simulink model "SIL_PID_vs_LeadLag"  (R2026a)
settings: Solver=VariableStepAuto
libraries: simulink_extras x14, simulink x4, slpidlib x2
settings Model: Creator=jamie  LastModifiedBy=root

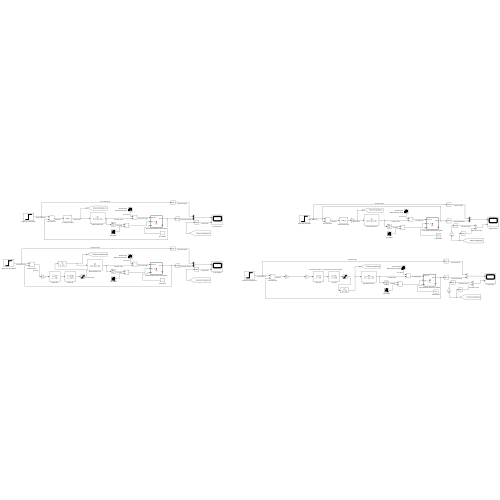
[thumbnail: Simulink's stored preview of the top-level diagram]
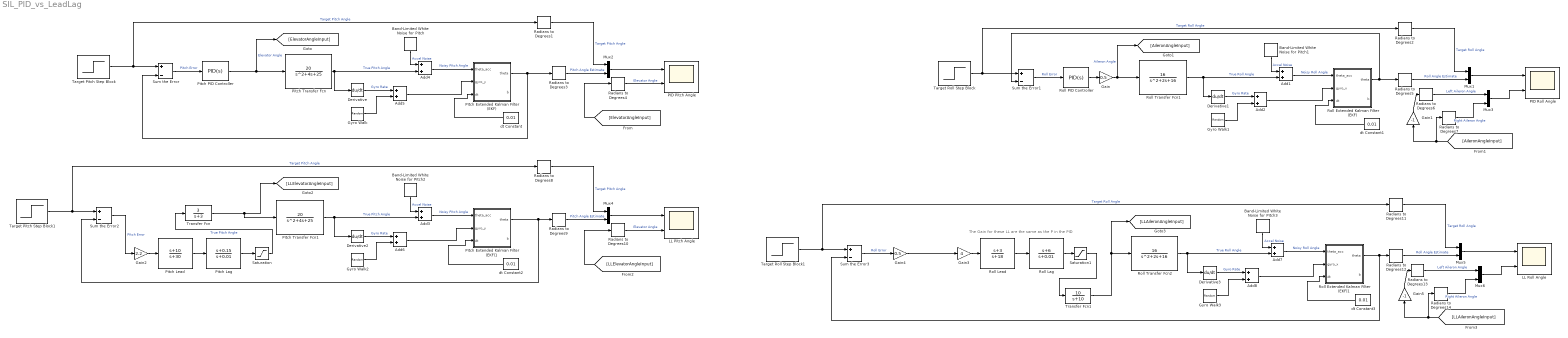
== system SIL_PID_vs_LeadLag ==
  note: The Gain for these LL are the same as the P in the PID
  Add{1..8} (8 alike) : Sum
  Band-Limited White Noise for Pitch : simulink/Sources/Band-Limited White Noise  Cov=[0 0.1]  Ts=0.01  seed=[23341]
  Band-Limited White Noise for Pitch1 : simulink/Sources/Band-Limited White Noise  Cov=[0 0.1]  Ts=0.01  seed=[23351]
  Band-Limited White Noise for Pitch2 : simulink/Sources/Band-Limited White Noise  Cov=[0 0.1]  Ts=0.01  seed=[23341]
  Band-Limited White Noise for Pitch3 : simulink/Sources/Band-Limited White Noise  Cov=[0 0.1]  Ts=0.01  seed=[23351]
  Derivative{,1..3} (4 alike) : Derivative
  Gain : Gain  Gain=0.5
  Gain1 : Gain  Gain=-1
  Gain2 : Gain  Gain=2.2
  Gain3 : Gain  Gain=4
  Gain4 : Gain  Gain=0.5
  Gain5 : Gain  Gain=-1
  Gyro Walk{,1..3} (4 alike) : RandomNumber  Mean=0.005  Variance=0.005  Seed=1324  SampleTime=0.01
  LL Pitch Angle : Scope  NumInputPorts=2
      settings: Title=Elevator Angle [Deg]  ActiveDisplayYMinimum=-0.78781696830479941  ActiveDisplayYMaximum=7.0903527147431964
  LL Roll Angle : Scope  NumInputPorts=2
      settings: Title=Aileron Angle [Deg]  ActiveDisplayYMinimum=-0.7819624383983379  ActiveDisplayYMaximum=6.7711261172971131  DataLoggingVariableName=ScopeData2
  Mux{1..6} (6 alike) : Mux  Inputs=2
  PID Pitch Angle : Scope  NumInputPorts=2
      settings: Title=Elevator Angle [Deg]  ActiveDisplayYMinimum=-14.441470160927292  ActiveDisplayYMaximum=71.717086630986358  DataLoggingVariableName=roll_data_LL
  PID Roll Angle : Scope  NumInputPorts=2
      settings: Title=Aileron Angle [Deg]  ActiveDisplayYMinimum=-0.73178120395973612  ActiveDisplayYMaximum=6.5860300050338685
  Pitch Extended Kalman Filter (EKF) : MATLAB Function  TreatAsAtomicUnit=on  SystemSampleTime=0.01
  Pitch Extended Kalman Filter (EKF)1 : MATLAB Function  TreatAsAtomicUnit=on  SystemSampleTime=0.01
  Pitch Lag : TransferFcn  Numerator=[1 0.15]  Denominator=[1 0.01]
  Pitch Lead : TransferFcn  Numerator=[1 10]  Denominator=[1 30]
  Pitch PID Controller : slpidlib/PID Controller  Controller=PID  Form=Parallel  TimeDomain=Continuous-time  UseExternalTs=off  SampleTime=-1  IntegratorMethod=Forward Euler  FilterMethod=Forward Euler  ControllerParametersSource=internal  P=4.0969544705731  I=10.602687289353  UseKiTs=off  D=0.285929702569769  UseExternalDerivativeSource=off  N=29.8204056271306  UseFilter=on  TunerSelectOption=Transfer Function Based (PID Tuner App)  InitialConditionSource=internal  InitialConditionForIntegrator=0  InitialConditionForFilter=0  DifferentiatorICPrevScaledInput=0  ExternalReset=none  TrackingMode=off  Kt=1  LimitOutput=off  SatLimitsSource=internal  UpperSaturationLimit=inf  LowerSaturationLimit=-inf  LinearizeAsGain=on  AntiWindupMode=none  Kb=1  LimitIntegrator=off  UpperIntegratorSaturationLimit=inf  LowerIntegratorSaturationLimit=-inf  POutMin=[]  POutMax=[]  IOutMin=[]  IOutMax=[]  DOutMin=[]  DOutMax=[]  NOutMin=[]  NOutMax=[]  SumOutMin=[]  SumOutMax=[]  SaturationOutMin=[]  SaturationOutMax=[]  PParamMin=[]  PParamMax=[]  IParamMin=[]  IParamMax=[]  DParamMin=[]  DParamMax=[]  NParamMin=[]  NParamMax=[]  KbParamMin=[]  KbParamMax=[]  KtParamMin=[]  KtParamMax=[]  KbOutMin=[]  KbOutMax=[]  KtOutMin=[]  KtOutMax=[]  IntegratorOutMin=[]  IntegratorOutMax=[]  FilterOutMin=[]  FilterOutMax=[]  SumI1OutMin=[]  SumI1OutMax=[]  SumI2OutMin=[]  SumI2OutMax=[]  SumI3OutMin=[]  SumI3OutMax=[]  SumI4OutMin=[]  SumI4OutMax=[]  SumDOutMin=[]  SumDOutMax=[]  DifferentiatorOutMin=[]  DifferentiatorOutMax=[]  FilterDiffOutCoefMin=[]  FilterDiffOutCoefMax=[]  ReciprocalOutMin=[]  ReciprocalOutMax=[]  SumDenOutMin=[]  SumDenOutMax=[]  SumNumOutMin=[]  SumNumOutMax=[]  DivideOutMin=[]  DivideOutMax=[]  UdiffTsProdOutMin=[]  UdiffTsProdOutMax=[]  NTsProdOutMin=[]  NTsProdOutMax=[]  UintegralTsProdOutMin=[]  UintegralTsProdOutMax=[]  UngainTsProdOutMin=[]  UngainTsProdOutMax=[]  ClampingZeroOutDataTypeStr=Inherit: Inherit via back propagation  ClampingZeroOutMin=[]  ClampingZeroOutMax=[]  FilterDenConstantOutDataTypeStr=Inherit: Inherit via back propagation  FilterDenConstantOutMin=[]  FilterDenConstantOutMax=[]  PCopyOutDataTypeStr=Inherit: Inherit via back propagation  PCopyOutMin=[]  PCopyOutMax=[]  NCopyOutDataTypeStr=Inherit: Inherit via back propagation  NCopyOutMin=[]  NCopyOutMax=[]  IntegratorContinuousStateAttributes=''  IntegratorStateMustResolveToSignalObject=off  IntegratorRTWStateStorageClass=Auto  FilterContinuousStateAttributes=''  FilterStateMustResolveToSignalObject=off  FilterRTWStateStorageClass=Auto  ParallelPVariant=InternalParameters  IdealPVariant=Disabled  IVariant=InternalParameters  DVariant=InternalParameters  IntegratorVariant=Continuous  SatVariant=Disabled  AWVariant=Passthrough  PCopyVariant=Disabled  TRVariant=Disabled  FdbkBlocksVariant=Forward  IdealPFdbkVariant=Disabled  SatFdbkVariant=Disabled  DerivativeFilterVariant=ContFilter  NVariant=InternalParameters  NCopyVariant=Disabled  FilterICVariant=InternalICsFilter  IntegratorICVariant=InternalICs  ExternalResetVariant=Disabled  TRSumVariant=Passthrough  SumFdbkVariant=Disabled  SumVariant=Sum_PID  TsampFilterVariant=InternalTs  TsampNgainVariant=Passthrough  TsampIntegralVariant=Disabled_SignalSpec  ExternalSaturationOutDataTypeStr=Inherit: Same as second input  DerivativeSourceVariant=ErrorSignal  PreIntVariant=InternalPreInt
  Pitch Transfer Fcn : TransferFcn  Numerator=[20]  Denominator=[1 4 25]
  Pitch Transfer Fcn1 : TransferFcn  Numerator=[20]  Denominator=[1 4 25]
  Radians to Degrees{1..14} (14 alike) : simulink_extras/Transformations/Radians to Degrees
  Roll Extended Kalman Filter (EKF) : MATLAB Function  TreatAsAtomicUnit=on  SystemSampleTime=0.01
  Roll Extended Kalman Filter (EKF)1 : MATLAB Function  TreatAsAtomicUnit=on  SystemSampleTime=0.01
  Roll Lag : TransferFcn  Numerator=[1 6]  Denominator=[1 0.01]
  Roll Lead : TransferFcn  Numerator=[1 3]  Denominator=[1 18]
  Roll PID Controller : slpidlib/PID Controller  Controller=PID  Form=Parallel  TimeDomain=Continuous-time  UseExternalTs=off  SampleTime=-1  IntegratorMethod=Forward Euler  FilterMethod=Forward Euler  ControllerParametersSource=internal  P=2  I=5  UseKiTs=off  D=0.1  UseExternalDerivativeSource=off  N=10  UseFilter=on  TunerSelectOption=Transfer Function Based (PID Tuner App)  InitialConditionSource=internal  InitialConditionForIntegrator=0  InitialConditionForFilter=0  DifferentiatorICPrevScaledInput=0  ExternalReset=none  TrackingMode=off  Kt=1  LimitOutput=off  SatLimitsSource=internal  UpperSaturationLimit=inf  LowerSaturationLimit=-inf  LinearizeAsGain=on  AntiWindupMode=none  Kb=1  LimitIntegrator=off  UpperIntegratorSaturationLimit=inf  LowerIntegratorSaturationLimit=-inf  POutMin=[]  POutMax=[]  IOutMin=[]  IOutMax=[]  DOutMin=[]  DOutMax=[]  NOutMin=[]  NOutMax=[]  SumOutMin=[]  SumOutMax=[]  SaturationOutMin=[]  SaturationOutMax=[]  PParamMin=[]  PParamMax=[]  IParamMin=[]  IParamMax=[]  DParamMin=[]  DParamMax=[]  NParamMin=[]  NParamMax=[]  KbParamMin=[]  KbParamMax=[]  KtParamMin=[]  KtParamMax=[]  KbOutMin=[]  KbOutMax=[]  KtOutMin=[]  KtOutMax=[]  IntegratorOutMin=[]  IntegratorOutMax=[]  FilterOutMin=[]  FilterOutMax=[]  SumI1OutMin=[]  SumI1OutMax=[]  SumI2OutMin=[]  SumI2OutMax=[]  SumI3OutMin=[]  SumI3OutMax=[]  SumI4OutMin=[]  SumI4OutMax=[]  SumDOutMin=[]  SumDOutMax=[]  DifferentiatorOutMin=[]  DifferentiatorOutMax=[]  FilterDiffOutCoefMin=[]  FilterDiffOutCoefMax=[]  ReciprocalOutMin=[]  ReciprocalOutMax=[]  SumDenOutMin=[]  SumDenOutMax=[]  SumNumOutMin=[]  SumNumOutMax=[]  DivideOutMin=[]  DivideOutMax=[]  UdiffTsProdOutMin=[]  UdiffTsProdOutMax=[]  NTsProdOutMin=[]  NTsProdOutMax=[]  UintegralTsProdOutMin=[]  UintegralTsProdOutMax=[]  UngainTsProdOutMin=[]  UngainTsProdOutMax=[]  ClampingZeroOutDataTypeStr=Inherit: Inherit via back propagation  ClampingZeroOutMin=[]  ClampingZeroOutMax=[]  FilterDenConstantOutDataTypeStr=Inherit: Inherit via back propagation  FilterDenConstantOutMin=[]  FilterDenConstantOutMax=[]  PCopyOutDataTypeStr=Inherit: Inherit via back propagation  PCopyOutMin=[]  PCopyOutMax=[]  NCopyOutDataTypeStr=Inherit: Inherit via back propagation  NCopyOutMin=[]  NCopyOutMax=[]  IntegratorContinuousStateAttributes=''  IntegratorStateMustResolveToSignalObject=off  IntegratorRTWStateStorageClass=Auto  FilterContinuousStateAttributes=''  FilterStateMustResolveToSignalObject=off  FilterRTWStateStorageClass=Auto  ParallelPVariant=InternalParameters  IdealPVariant=Disabled  IVariant=InternalParameters  DVariant=InternalParameters  IntegratorVariant=Continuous  SatVariant=Disabled  AWVariant=Passthrough  PCopyVariant=Disabled  TRVariant=Disabled  FdbkBlocksVariant=Forward  IdealPFdbkVariant=Disabled  SatFdbkVariant=Disabled  DerivativeFilterVariant=ContFilter  NVariant=InternalParameters  NCopyVariant=Disabled  FilterICVariant=InternalICsFilter  IntegratorICVariant=InternalICs  ExternalResetVariant=Disabled  TRSumVariant=Passthrough  SumFdbkVariant=Disabled  SumVariant=Sum_PID  TsampFilterVariant=InternalTs  TsampNgainVariant=Passthrough  TsampIntegralVariant=Disabled_SignalSpec  ExternalSaturationOutDataTypeStr=Inherit: Same as second input  DerivativeSourceVariant=ErrorSignal  PreIntVariant=InternalPreInt
  Roll Transfer Fcn1 : TransferFcn  Numerator=[16]  Denominator=[1 2 16]
  Roll Transfer Fcn2 : TransferFcn  Numerator=[16]  Denominator=[1 2 16]
  Saturation : Saturate  UpperLimit=0.11  LowerLimit=0.11
  Saturation1 : Saturate  UpperLimit=0.088  LowerLimit=-0.088
  Sum the Error{,1..3} (4 alike) : Sum  Inputs=+-
  Target Pitch Step Block : Step  Time=0.01  FinalValue=0.087266  SampleTime=0
  Target Pitch Step Block1 : Step  Time=0.01  FinalValue=0.087266  SampleTime=0
  Target Roll Step Block : Step  Time=0.01  FinalValue=0.087266  SampleTime=0
  Target Roll Step Block1 : Step  Time=0.01  FinalValue=0.087266  SampleTime=0
  Transfer Fcn : TransferFcn  Numerator=[3]  Denominator=[1 3]
  Transfer Fcn1 : TransferFcn  Numerator=[10]  Denominator=[1 10]
  dt Constant{,1..3} (4 alike) : Constant  Value=0.01
  wires:
  Pitch PID Controller/1 -> Pitch Transfer Fcn/1, [ElevatorAngleInput]  "Elevator Angle"
  dt Constant/1 -> Pitch Extended Kalman Filter (EKF)/3(dt)
  Add4/1 -> Pitch Extended Kalman Filter (EKF)/1(theta_acc)  "Noisy Pitch Angle"
  Pitch Transfer Fcn/1 -> Add4/2, Derivative/1  "True Pitch Angle"
  Band-Limited White Noise for Pitch/1 -> Add4/1  "Accel Noise"
  Derivative/1 -> Add5/1  "Gyro Rate"
  Gyro Walk/1 -> Add5/2
  Add5/1 -> Pitch Extended Kalman Filter (EKF)/2(gyro_y)
  Sum the Error/1 -> Pitch PID Controller/1  "Pitch Error"
  Target Pitch Step Block/1 -> Radians to Degrees1/1, Sum the Error/1  "Target Pitch Angle"
  Pitch Extended Kalman Filter (EKF)/1(theta) -> Radians to Degrees3/1, Sum the Error/2
  [ElevatorAngleInput] -> Radians to Degrees4/1
  Mux2/1 -> PID Pitch Angle/1
  Radians to Degrees3/1 -> Mux2/2  "Pitch Angle Estimate"
  Radians to Degrees1/1 -> Mux2/1  "Target Pitch Angle"
  Radians to Degrees4/1 -> PID Pitch Angle/2  "Elevator Angle"
  Derivative1/1 -> Add2/1  "Gyro Rate"
  Gyro Walk1/1 -> Add2/2
  [AileronAngleInput] -> Gain1/1, Radians to Degrees7/1
  Roll PID Controller/1 -> Gain/1
  Roll Extended Kalman Filter (EKF)/1(theta) -> Radians to Degrees5/1, Sum the Error1/2
  Target Roll Step Block/1 -> Radians to Degrees2/1, Sum the Error1/1  "Target Roll Angle"
  Radians to Degrees5/1 -> Mux1/2  "Roll Angle Estimate"
  Mux1/1 -> PID Roll Angle/1
  dt Constant1/1 -> Roll Extended Kalman Filter (EKF)/3(dt)
  Add1/1 -> Roll Extended Kalman Filter (EKF)/1(theta_acc)  "Noisy Roll Angle"
  Band-Limited White Noise for Pitch1/1 -> Add1/1  "Accel Noise"
  Sum the Error1/1 -> Roll PID Controller/1  "Roll Error"
  Add2/1 -> Roll Extended Kalman Filter (EKF)/2(gyro_x)
  Roll Transfer Fcn1/1 -> Add1/2, Derivative1/1  "True Roll Angle"
  Radians to Degrees2/1 -> Mux1/1  "Target Roll Angle"
  Gain/1 -> Roll Transfer Fcn1/1, [AileronAngleInput]  "Aileron Angle"
  Mux3/1 -> PID Roll Angle/2
  Radians to Degrees7/1 -> Mux3/2  "Right Aileron Angle"
  Radians to Degrees6/1 -> Mux3/1  "Left Aileron Angle"
  Gain1/1 -> Radians to Degrees6/1
  Derivative2/1 -> Add6/1  "Gyro Rate"
  Gyro Walk2/1 -> Add6/2
  [LLElevatorAngleInput] -> Radians to Degrees10/1
  Pitch Extended Kalman Filter (EKF)1/1(theta) -> Radians to Degrees9/1, Sum the Error2/2
  Target Pitch Step Block1/1 -> Radians to Degrees8/1, Sum the Error2/1  "Target Pitch Angle"
  Radians to Degrees9/1 -> Mux4/2  "Pitch Angle Estimate"
  Mux4/1 -> LL Pitch Angle/1
  Radians to Degrees10/1 -> LL Pitch Angle/2  "Elevator Angle"
  dt Constant2/1 -> Pitch Extended Kalman Filter (EKF)1/3(dt)
  Add3/1 -> Pitch Extended Kalman Filter (EKF)1/1(theta_acc)  "Noisy Pitch Angle"
  Band-Limited White Noise for Pitch2/1 -> Add3/1  "Accel Noise"
  Sum the Error2/1 -> Gain2/1  "Pitch Error"
  Add6/1 -> Pitch Extended Kalman Filter (EKF)1/2(gyro_y)
  Pitch Transfer Fcn1/1 -> Add3/2, Derivative2/1  "True Pitch Angle"
  Radians to Degrees8/1 -> Mux4/1  "Target Pitch Angle"
  Roll Lag/1 -> Saturation1/1
  Pitch Lag/1 -> Saturation/1
  Pitch Lead/1 -> Pitch Lag/1
  Gain2/1 -> Pitch Lead/1
  Gain3/1 -> Roll Lead/1
  Roll Lead/1 -> Roll Lag/1
  Gyro Walk3/1 -> Add8/2
  Add8/1 -> Roll Extended Kalman Filter (EKF)1/2(gyro_x)
  Gain5/1 -> Radians to Degrees13/1
  Roll Extended Kalman Filter (EKF)1/1(theta) -> Radians to Degrees12/1, Sum the Error3/2
  Band-Limited White Noise for Pitch3/1 -> Add7/1  "Accel Noise"
  Sum the Error3/1 -> Gain4/1  "Roll Error"
  Add7/1 -> Roll Extended Kalman Filter (EKF)1/1(theta_acc)  "Noisy Roll Angle"
  dt Constant3/1 -> Roll Extended Kalman Filter (EKF)1/3(dt)
  Derivative3/1 -> Add8/1  "Gyro Rate"
  Radians to Degrees12/1 -> Mux5/2  "Roll Angle Estimate"
  Target Roll Step Block1/1 -> Radians to Degrees11/1, Sum the Error3/1  "Target Roll Angle"
  Radians to Degrees14/1 -> Mux6/2  "Right Aileron Angle"
  [LLAileronAngleInput] -> Gain5/1, Radians to Degrees14/1
  Radians to Degrees11/1 -> Mux5/1  "Target Roll Angle"
  Mux5/1 -> LL Roll Angle/1
  Radians to Degrees13/1 -> Mux6/1  "Left Aileron Angle"
  Mux6/1 -> LL Roll Angle/2
  Roll Transfer Fcn2/1 -> Add7/2, Derivative3/1  "True Roll Angle"
  Gain4/1 -> Gain3/1
  Transfer Fcn/1 -> [LLElevatorAngleInput], Pitch Transfer Fcn1/1
  Saturation/1 -> Transfer Fcn/1  "True Pitch Angle"
  Transfer Fcn1/1 -> Roll Transfer Fcn2/1, [LLAileronAngleInput]
  Saturation1/1 -> Transfer Fcn1/1

== matlab function SIL_PID_vs_LeadLag/Roll Extended Kalman Filter (EKF) ==
  data: theta_acc input; theta output; gyro_x input; dt input; b output
function [theta, b] = fcn(theta_acc, gyro_x, dt)
    % Force inputs to double precision
    theta_acc = double(theta_acc);
    gyro_x    = double(gyro_x);
    dt        = double(dt);

    persistent x P
    if isempty(x)
        x = [0; 0];    % Explicit 2x1 column vector
        P = eye(2);    % Explicit 2x2 identity matrix
    end

    % Empirical Covariances
    R = 0.00000382;
    Q = [4.0e-10 , 0 ;
         0       , 1.0e-6];

    % System Matrices
    A = [1, -dt; 0, 1];
    B = [dt; 0];

    % 1. Predict Step
    x_pred = A * x + B * gyro_x;
    P_pred = A * P * A' + Q;

    % 2. Non-linear Measurement Update
    H = [cos(x_pred(1)), 0];
    
    % EXPLICIT SCALAR CASTING FOR Y_TILDE
    y_tilde = double(sin(theta_acc) - sin(x_pred(1)));
    y_tilde = y_tilde(1); % Hard-guarantee 1x1 scalar dimension

    % Compute Kalman Gain (2x1)
    S = H * P_pred * H' + R;
    K = (P_pred * H') / S;

    % State and Covariance Updates
    x = x_pred + K * y_tilde;
    P = (eye(2) - K * H) * P_pred;

    % Clamp pitch angle to [-pi, pi]
    x(1) = atan2(sin(x(1)), cos(x(1)));

    % Explicit Scalar Output Assignments
    theta = double(x(1));
    b     = double(x(2));
end

== matlab function SIL_PID_vs_LeadLag/Pitch Extended Kalman Filter (EKF)1 ==
  data: theta_acc input; theta output; gyro_y input; dt input; b output
function [theta, b] = fcn(theta_acc, gyro_y, dt)
    % Force inputs to double precision
    theta_acc = double(theta_acc);
    gyro_y    = double(gyro_y);
    dt        = double(dt);

    persistent x P
    if isempty(x)
        x = [0; 0];    % Explicit 2x1 column vector
        P = eye(2);    % Explicit 2x2 identity matrix
    end

    % Empirical Covariances
    R = 0.00000382;
    Q = [4.0e-10 , 0 ;
         0       , 1.0e-6];

    % System Matrices
    A = [1, -dt; 0, 1];
    B = [dt; 0];

    % 1. Predict Step
    x_pred = A * x + B * gyro_y;
    P_pred = A * P * A' + Q;

    % 2. Non-linear Measurement Update
    H = [cos(x_pred(1)), 0];
    
    % EXPLICIT SCALAR CASTING FOR Y_TILDE
    y_tilde = double(sin(theta_acc) - sin(x_pred(1)));
    y_tilde = y_tilde(1); % Hard-guarantee 1x1 scalar dimension

    % Compute Kalman Gain (2x1)
    S = H * P_pred * H' + R;
    K = (P_pred * H') / S;

    % State and Covariance Updates
    x = x_pred + K * y_tilde;
    P = (eye(2) - K * H) * P_pred;

    % Clamp pitch angle to [-pi, pi]
    x(1) = atan2(sin(x(1)), cos(x(1)));

    % Explicit Scalar Output Assignments
    theta = double(x(1));
    b     = double(x(2));
end

== matlab function SIL_PID_vs_LeadLag/Roll Extended Kalman Filter (EKF)1 ==
  data: theta_acc input; theta output; gyro_x input; dt input; b output
function [theta, b] = fcn(theta_acc, gyro_x, dt)
    % Force inputs to double precision
    theta_acc = double(theta_acc);
    gyro_x    = double(gyro_x);
    dt        = double(dt);

    persistent x P
    if isempty(x)
        x = [0; 0];    % Explicit 2x1 column vector
        P = eye(2);    % Explicit 2x2 identity matrix
    end

    % Empirical Covariances
    R = 0.00000382;
    Q = [4.0e-10 , 0 ;
         0       , 1.0e-6];

    % System Matrices
    A = [1, -dt; 0, 1];
    B = [dt; 0];

    % 1. Predict Step
    x_pred = A * x + B * gyro_x;
    P_pred = A * P * A' + Q;

    % 2. Non-linear Measurement Update
    H = [cos(x_pred(1)), 0];
    
    % EXPLICIT SCALAR CASTING FOR Y_TILDE
    y_tilde = double(sin(theta_acc) - sin(x_pred(1)));
    y_tilde = y_tilde(1); % Hard-guarantee 1x1 scalar dimension

    % Compute Kalman Gain (2x1)
    S = H * P_pred * H' + R;
    K = (P_pred * H') / S;

    % State and Covariance Updates
    x = x_pred + K * y_tilde;
    P = (eye(2) - K * H) * P_pred;

    % Clamp pitch angle to [-pi, pi]
    x(1) = atan2(sin(x(1)), cos(x(1)));

    % Explicit Scalar Output Assignments
    theta = double(x(1));
    b     = double(x(2));
end

== matlab function SIL_PID_vs_LeadLag/Pitch Extended Kalman Filter (EKF) ==
  data: theta_acc input; theta output; gyro_y input; dt input; b output
function [theta, b] = fcn(theta_acc, gyro_y, dt)
    % Force inputs to double precision
    theta_acc = double(theta_acc);
    gyro_y    = double(gyro_y);
    dt        = double(dt);

    persistent x P
    if isempty(x)
        x = [0; 0];    % Explicit 2x1 column vector
        P = eye(2);    % Explicit 2x2 identity matrix
    end

    % Empirical Covariances
    R = 0.00000382;
    Q = [4.0e-10 , 0 ;
         0       , 1.0e-6];

    % System Matrices
    A = [1, -dt; 0, 1];
    B = [dt; 0];

    % 1. Predict Step
    x_pred = A * x + B * gyro_y;
    P_pred = A * P * A' + Q;

    % 2. Non-linear Measurement Update
    H = [cos(x_pred(1)), 0];
    
    % EXPLICIT SCALAR CASTING FOR Y_TILDE
    y_tilde = double(sin(theta_acc) - sin(x_pred(1)));
    y_tilde = y_tilde(1); % Hard-guarantee 1x1 scalar dimension

    % Compute Kalman Gain (2x1)
    S = H * P_pred * H' + R;
    K = (P_pred * H') / S;

    % State and Covariance Updates
    x = x_pred + K * y_tilde;
    P = (eye(2) - K * H) * P_pred;

    % Clamp pitch angle to [-pi, pi]
    x(1) = atan2(sin(x(1)), cos(x(1)));

    % Explicit Scalar Output Assignments
    theta = double(x(1));
    b     = double(x(2));
end
